simulink model "demoOtterUSVPathFollowingHeadingControl"  (R2024a)
settings: Solver=ode4  StartTime=0.0  StopTime=1200  FixedStep=0.05  RelTol=1e-3
libraries: mssSimulink x6
settings Model: Creator=thor  LastModifiedBy=thor
settings DataIOCC: ReturnWorkspaceOutputs=off
settings DebuggingCC: UnconnectedInputMsg=warning  UnconnectedOutputMsg=warning  UnconnectedLineMsg=warning
settings ModelReferenceCC: EnableRefExpFcnMdlSchedulingChecks=on
settings RTWCC: GPUComputeCapability=3.5  DLArmComputeVersion=19.05

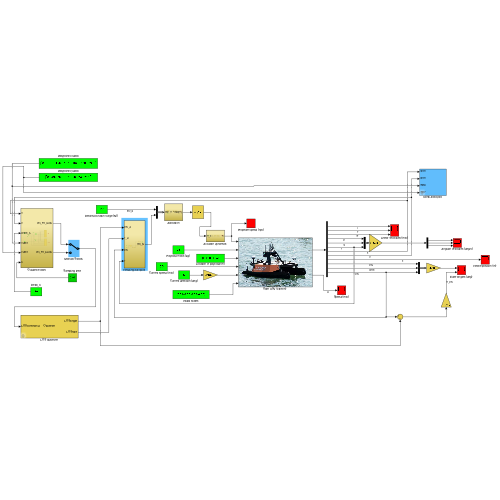
[thumbnail: Simulink's stored preview of the top-level diagram]
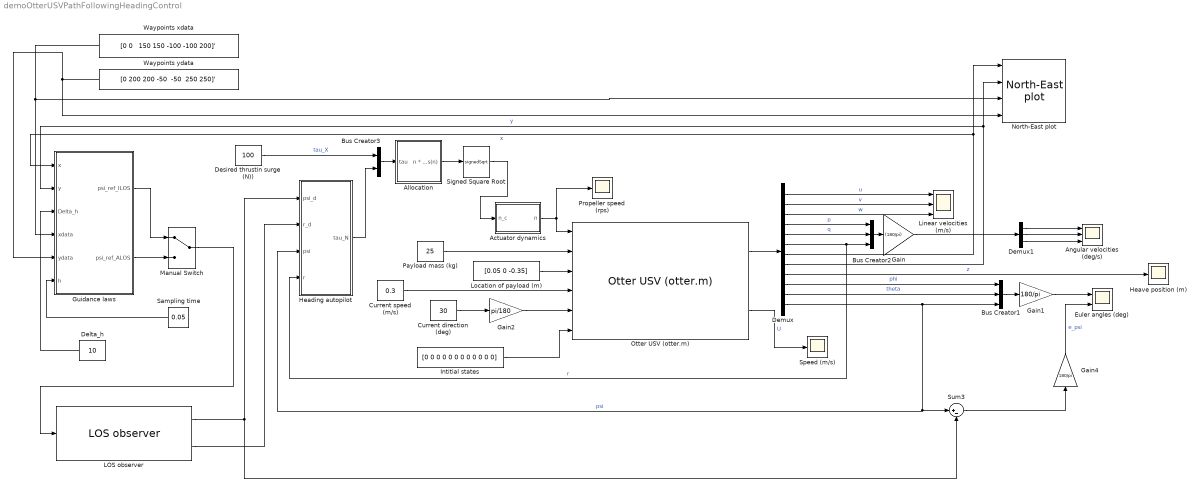
== system demoOtterUSVPathFollowingHeadingControl ==
  Actuator dynamics : Subsystem
  Allocation : Subsystem
  Angular velocities (deg/s) : Scope  NumInputPorts=3
  Bus Creator1 : BusCreator  Inputs=3
  Bus Creator2 : BusCreator  Inputs=3
  Bus Creator3 : BusCreator  Inputs=2
  Current direction (deg) : Constant  Value=30
  Current speed (m/s) : Constant  Value=0.3
  Delta_h : Constant  Value=10
  Demux : Demux  Outputs=12
  Demux1 : Demux  Outputs=3
  Desired thrustin surge (N)) : Constant  Value=100
  Euler angles (deg) : Scope  NumInputPorts=2
  Gain : Gain  Gain=(180/pi)
  Gain1 : Gain  Gain=180/pi
  Gain2 : Gain  Gain=pi/180
  Gain4 : Gain  Gain=180/pi
  Guidance laws : Subsystem
  Heading autopilot : Subsystem
  Heave position (m) : Scope
  Intitial states : Constant  Value=[0 0 0 0 0 0 0 0 0 0 0 0]
  LOS observer : mssSimulink/Guidance/LOS observer  K_f=0.3  alpha=5
  Linear velocities (m/s) : Scope  NumInputPorts=3
  Location of payload (m) : Constant  Value=[0.05 0 -0.35]
  Manual Switch : ManualSwitch
  North-East plot : mssSimulink/Utilities/Visualization/North-East plot  decimation=10
  "Otter USV (otter.m) " : mssSimulink/Marine craft models/Otter USV (otter.m)  SystemSampleTime=-1  VariantActivationTime=update diagram  AllowFlexibleInterface=on  Latency=0  AutoFrameSizeCalculation=off
  Payload mass (kg) : Constant  Value=25
  Propeller speed (rps) : Scope
  Sampling time : Constant  Value=0.05
  Signed Square Root : Sqrt  Operator=signedSqrt
  Speed (m/s) : Scope
  Sum3 : Sum  Inputs=|+-  InputSameDT=on  SaturateOnIntegerOverflow=on  OutDataTypeStr=Inherit: Same as first input
  Waypoints xdata : Constant  Value="[0 0   150 150 -100 -100 200]'"
  Waypoints ydata : Constant  Value="[0 200 200 -50  -50  250 250]'"
  wires:
  Demux/1 -> Linear velocities (m/s)/1  "u"
  Demux/2 -> Linear velocities (m/s)/2  "v"
  Demux/3 -> Linear velocities (m/s)/3  "w"
  Demux/10 -> Bus Creator1/1  "phi"
  Demux/11 -> Bus Creator1/2  "theta"
  Demux/4 -> Bus Creator2/1  "p"
  Demux/5 -> Bus Creator2/2  "q"
  Demux/9 -> Heave position (m)/1  "z"
  Payload mass (kg)/1 -> "Otter USV (otter.m) "/2
  Location of payload (m)/1 -> "Otter USV (otter.m) "/3
  Current speed (m/s)/1 -> "Otter USV (otter.m) "/4
  Current direction (deg)/1 -> Gain2/1
  Intitial states/1 -> "Otter USV (otter.m) "/6
  "Otter USV (otter.m) "/1 -> Demux/1
  Gain1/1 -> Euler angles (deg)/1
  Gain2/1 -> "Otter USV (otter.m) "/5
  Heading autopilot/1(tau_N) -> Bus Creator3/2
  Demux/6 -> Bus Creator2/3, Heading autopilot/4(r)  "r"
  Desired thrustin surge (N))/1 -> Bus Creator3/1  "tau_X"
  Bus Creator3/1 -> Allocation/1(tau)
  Bus Creator1/1 -> Gain1/1
  Demux/7 -> North-East plot/1, Guidance laws/1(x)  "x"
  Demux/12 -> Bus Creator1/3, Heading autopilot/3(psi), Sum3/1  "psi"
  Allocation/1(n * abs(n)) -> Signed Square Root/1
  Sum3/1 -> Gain4/1
  Gain4/1 -> Euler angles (deg)/2  "e_psi"
  "Otter USV (otter.m) "/2 -> Speed (m/s)/1  "U"
  Demux/8 -> North-East plot/2, Guidance laws/2(y)  "y"
  Guidance laws/1(psi_ref_ILOS) -> Manual Switch/1
  Guidance laws/2(psi_ref_ALOS) -> Manual Switch/2
  Actuator dynamics/1(n) -> Propeller speed (rps)/1, "Otter USV (otter.m) "/1
  Signed Square Root/1 -> Actuator dynamics/1(n_c)
  LOS observer/1 -> Sum3/2, Heading autopilot/1(psi_d)
  LOS observer/2 -> Heading autopilot/2(r_d)
  Manual Switch/1 -> LOS observer/1
  Waypoints ydata/1 -> North-East plot/4, Guidance laws/5(ydata)
  Waypoints xdata/1 -> Guidance laws/4(xdata), North-East plot/3
  Delta_h/1 -> Guidance laws/3(Delta_h)
  Sampling time/1 -> Guidance laws/6(h)
  Bus Creator2/1 -> Gain/1
  Gain/1 -> Demux1/1
  Demux1/1 -> Angular velocities (deg/s)/1
  Demux1/3 -> Angular velocities (deg/s)/3
  Demux1/2 -> Angular velocities (deg/s)/2

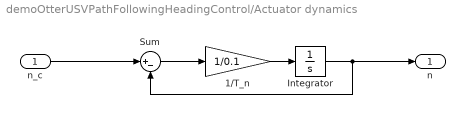
== system demoOtterUSVPathFollowingHeadingControl/Actuator dynamics ==
  n_c : Inport
  1/T_n : Gain  Gain=1/0.1
  Integrator : Integrator
  Sum : Sum  Inputs=|+-
  n : Outport
  wires:
  1/T_n/1 -> Integrator/1
  Integrator/1 -> n/1, Sum/2
  n_c/1 -> Sum/1
  Sum/1 -> 1/T_n/1

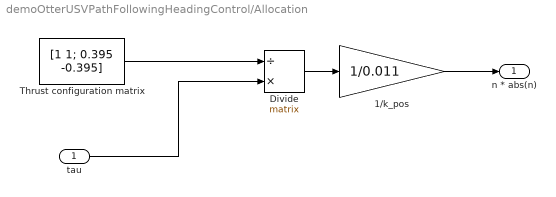
== system demoOtterUSVPathFollowingHeadingControl/Allocation ==
  tau : Inport
  1/k_pos : Gain  Gain=1/0.011
  Divide : Product  Inputs=/*  Multiplication=Matrix(*)
  Thrust configuration matrix : Constant  Value=[1 1; 0.395 -0.395]
  n * abs(n) : Outport
  wires:
  1/k_pos/1 -> n * abs(n)/1
  tau/1 -> Divide/2
  Divide/1 -> 1/k_pos/1
  Thrust configuration matrix/1 -> Divide/1

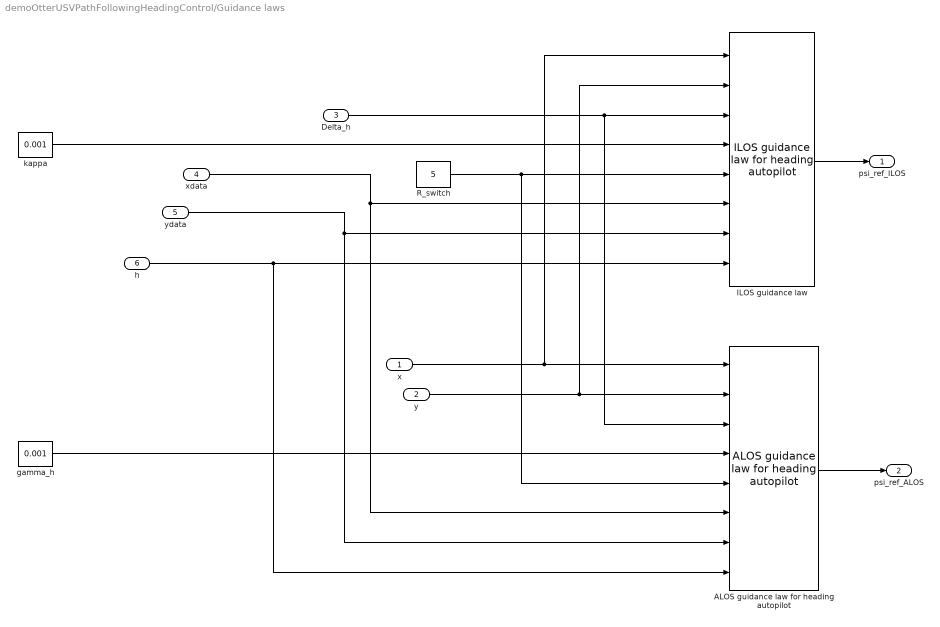
== system demoOtterUSVPathFollowingHeadingControl/Guidance laws ==
  x : Inport
  y : Inport  Port=2
  Delta_h : Inport  Port=3
  xdata : Inport  Port=4
  ydata : Inport  Port=5
  h : Inport  Port=6
  ALOS guidance law for heading autopilot : mssSimulink/Guidance/ALOS guidance law for heading autopilot  SystemSampleTime=-1  VariantActivationTime=update diagram  AllowFlexibleInterface=on  Latency=0  AutoFrameSizeCalculation=off
  ILOS guidance law : mssSimulink/Guidance/ILOS guidance law for heading autopilot  SystemSampleTime=-1  VariantActivationTime=update diagram  AllowFlexibleInterface=on  Latency=0  AutoFrameSizeCalculation=off
  R_switch : Constant  Value=5
  gamma_h : Constant  Value=0.001
  kappa : Constant  Value=0.001
  psi_ref_ILOS : Outport
  psi_ref_ALOS : Outport  Port=2
  wires:
  ILOS guidance law/1 -> psi_ref_ILOS/1
  gamma_h/1 -> ALOS guidance law for heading autopilot/4
  R_switch/1 -> ALOS guidance law for heading autopilot/5, ILOS guidance law/5
  h/1 -> ILOS guidance law/8, ALOS guidance law for heading autopilot/8
  y/1 -> ILOS guidance law/2, ALOS guidance law for heading autopilot/2
  ydata/1 -> ALOS guidance law for heading autopilot/7, ILOS guidance law/7
  kappa/1 -> ILOS guidance law/4
  x/1 -> ILOS guidance law/1, ALOS guidance law for heading autopilot/1
  ALOS guidance law for heading autopilot/1 -> psi_ref_ALOS/1
  Delta_h/1 -> ILOS guidance law/3, ALOS guidance law for heading autopilot/3
  xdata/1 -> ALOS guidance law for heading autopilot/6, ILOS guidance law/6

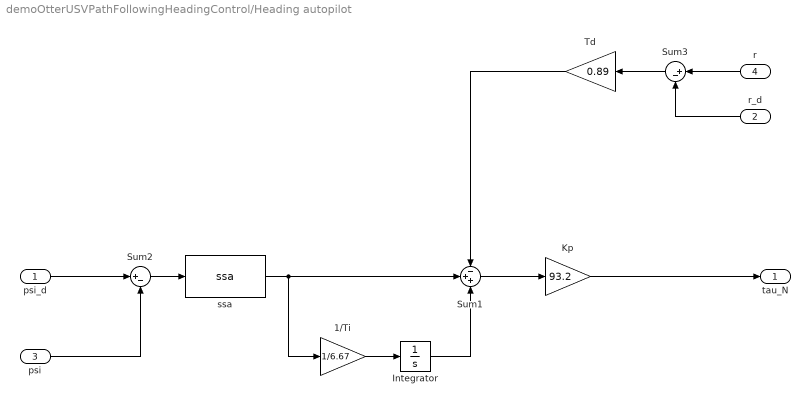
== system demoOtterUSVPathFollowingHeadingControl/Heading autopilot ==
  psi_d : Inport
  r_d : Inport  Port=2
  psi : Inport  Port=3
  r : Inport  Port=4
  1/Ti : Gain  Gain=1/6.67  SaturateOnIntegerOverflow=on  OutDataTypeStr=Inherit: Same as input  ParamDataTypeStr=Inherit: Same as input
  Integrator : Integrator
  Kp : Gain  Gain=93.2  SaturateOnIntegerOverflow=on  OutDataTypeStr=Inherit: Same as input  ParamDataTypeStr=Inherit: Same as input
  Sum1 : Sum  Inputs=-++  InputSameDT=on  SaturateOnIntegerOverflow=on  OutDataTypeStr=Inherit: Same as first input
  Sum2 : Sum  Inputs=|+-  InputSameDT=on  SaturateOnIntegerOverflow=on  OutDataTypeStr=Inherit: Same as first input
  Sum3 : Sum  Inputs=|+-  InputSameDT=on  SaturateOnIntegerOverflow=on  OutDataTypeStr=Inherit: Same as first input
  Td : Gain  Gain=0.89  SaturateOnIntegerOverflow=on  OutDataTypeStr=Inherit: Same as input  ParamDataTypeStr=Inherit: Same as input
  "ssa " : mssSimulink/Utilities/Math Operations/ssa  SystemSampleTime=-1  VariantActivationTime=update diagram  AllowFlexibleInterface=on  Latency=0  AutoFrameSizeCalculation=off
  tau_N : Outport
  wires:
  Td/1 -> Sum1/1
  r/1 -> Sum3/1
  psi/1 -> Sum2/2
  psi_d/1 -> Sum2/1
  Sum2/1 -> "ssa "/1
  Sum1/1 -> Kp/1
  "ssa "/1 -> 1/Ti/1, Sum1/2
  1/Ti/1 -> Integrator/1
  Integrator/1 -> Sum1/3
  Sum3/1 -> Td/1
  Kp/1 -> tau_N/1
  r_d/1 -> Sum3/2
